simulink model "MSF_Proyecto_Angel_Montano_Rodriguez"  (R2024b)
settings: Solver=ode15s  StartTime=0.0  StopTime=10.0  MaxStep=1e-3  RelTol=1e-6  AbsTol=1e-10
libraries: fl_lib x18, nesl_utility x6, slpidlib x1
settings Model: Creator=ASUS  LastModifiedBy=ASUS
settings DataIOCC: SaveOutput=off  SignalLogging=off  DSMLogging=off  ReturnWorkspaceOutputs=off  TimeSaveName=t
settings DebuggingCC: AlgebraicLoopMsg=none  ArtificialAlgebraicLoopMsg=none  MaxConsecutiveZCsMsg=none  OperatingPointInterfaceChecksumMismatchMsg=none

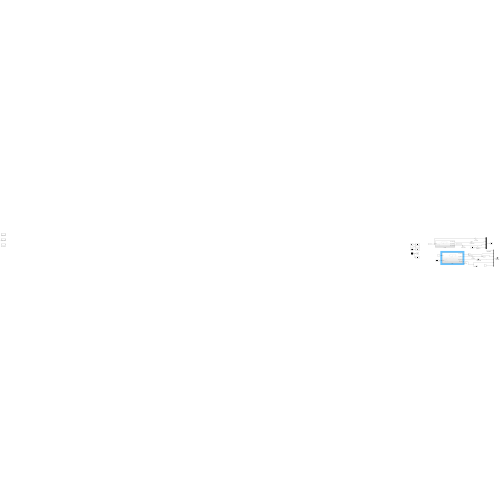
[thumbnail: Simulink's stored preview of the top-level diagram]
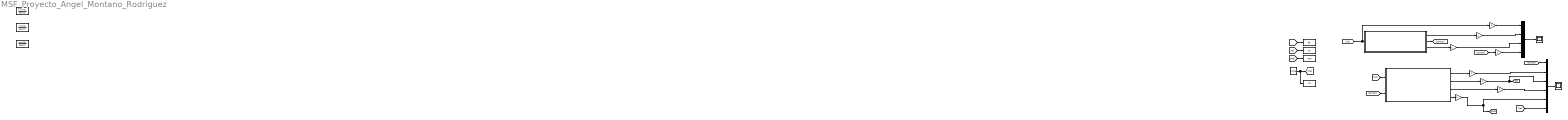
== system MSF_Proyecto_Angel_Montano_Rodriguez ==
  " Pp(t):Hipertenso" : TransferFcn  Numerator=[0.001,0.01]  Denominator=[0.00001,0.00101,0.01]
  " Pp(t):Hipotenso" : TransferFcn  Numerator=[0.001,0.01]  Denominator=[3.5E-5,0.00101,0.01]
  " Pp(t):Normotenso" : TransferFcn  Numerator=[0.001,0.01]  Denominator=[1.5E-5,0.00101,0.01]
  Caso : Subsystem
  Control : Subsystem
  EID(t): Control : Gain
  F(t): Caso CE : Gain
  F(t): Caso FT : Gain
  F(t): Control CE : Gain
  F(t): Control FT : Gain
  Mux2 : Mux  Inputs=6
  Mux3 : Mux
  PID(t): Caso : Gain
  Scope: Caso : Scope
  Scope: Control : Scope
  To Workspace1 : ToWorkspace  VariableName=Fe  SampleTime=-1
  To Workspace2 : ToWorkspace  VariableName=Fs  SampleTime=-1
  To Workspace3 : ToWorkspace  VariableName=PID  SampleTime=-1
  To Workspace4 : ToWorkspace  VariableName=Ve  SampleTime=-1
  Ve(t) : DiscretePulseGenerator  PulseType=Time based  Period=10  PulseWidth=10  PhaseDelay=1
  Ve(t) Control : Gain
  Ve(t): Caso EID : Gain
  wires:
  EID(t): Control/1 -> Mux3/3
  Mux3/1 -> Scope: Control/1
  F(t): Control CE/1 -> Mux3/2
  F(t): Control FT/1 -> Mux3/4
  F(t): Caso CE/1 -> Mux2/2
  Caso/1(Vs(t): Caso CE) -> F(t): Caso CE/1
  PID(t): Caso/1 -> Mux2/5, [PID]
  Mux2/1 -> Scope: Caso/1
  Caso/3(Ve(t): Caso EID) -> Ve(t): Caso EID/1
  Caso/4(PID(t): Caso) -> PID(t): Caso/1
  Ve(t)/1 -> To Workspace4/1, [Ve]
  [control] -> To Workspace1/1
  [Fs] -> To Workspace2/1
  [PID] -> To Workspace3/1
  Control/3(Ve(t): Control EID) -> EID(t): Control/1
  [control] -> F(t): Control FT/1
  Ve(t): Caso EID/1 -> Mux2/4
  Control/2(Ve(t): Control FT) -> [control]
  Control/1(Ve(t): Control CE) -> F(t): Control CE/1
  Caso/2(Ve(t): Caso FT) -> F(t): Caso FT/1
  [Ve] -> Ve(t) Control/1, Control/1(Ve(t))
  Ve(t) Control/1 -> Mux3/1
  [Ve] -> Caso/1(Vs(t))
  [control] -> Caso/2(Control)
  [Ve] -> Mux2/6
  [control] -> Mux2/1
  F(t): Caso FT/1 -> Mux2/3, [Fs]

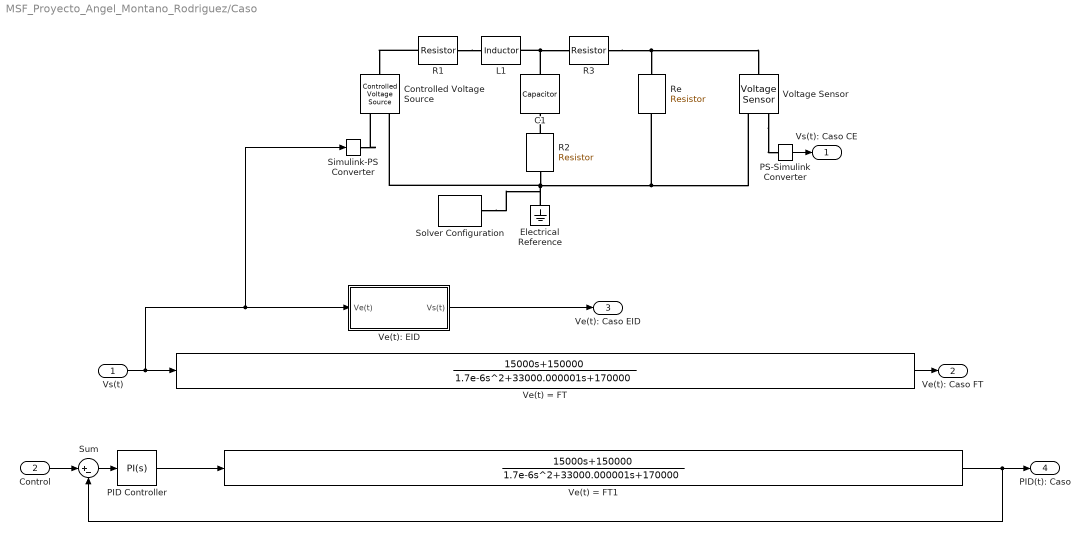
== system MSF_Proyecto_Angel_Montano_Rodriguez/Caso ==
  Vs(t) : Inport
  Control : Inport  Port=2
  " Ve(t) = FT" : TransferFcn  Numerator=[15000 150000]  Denominator=[1.7e-6 33000.000001 170000]
  " Ve(t) = FT1" : TransferFcn  Numerator=[15000 150000]  Denominator=[1.7e-6 33000.000001 170000]
  C1 : fl_lib/Electrical/Electrical Elements/Capacitor  c=10e-6 F  r=1e-6 Ohm  g=0 1/Ohm  i_specify=off  i_priority=None  i=0 A  i_nominal_specify=off  i_nominal_value=1  i_nominal_unit=A  v_specify=off  v_priority=None  v=0 V  v_nominal_specify=off  v_nominal_value=1  v_nominal_unit=V  vc_specify=off  vc_priority=High  vc=0 V  vc_nominal_specify=off  vc_nominal_value=1  vc_nominal_unit=V
  Controlled Voltage Source : fl_lib/Electrical/Electrical Sources/Controlled Voltage Source
  Electrical Reference : fl_lib/Electrical/Electrical Elements/Electrical Reference
  L1 : fl_lib/Electrical/Electrical Elements/Inductor  l=1e-6 H  r=0 Ohm  g=1e-9 1/Ohm  i_specify=off  i_priority=None  i=0 A  i_nominal_specify=off  i_nominal_value=1  i_nominal_unit=A  v_specify=off  v_priority=None  v=0 V  v_nominal_specify=off  v_nominal_value=1  v_nominal_unit=V  i_L_specify=off  i_L_priority=High  i_L=0 A  i_L_nominal_specify=off  i_L_nominal_value=1  i_L_nominal_unit=A
  PID Controller : slpidlib/PID Controller  Controller=PI  Form=Parallel  TimeDomain=Continuous-time  UseExternalTs=off  SampleTime=-1  IntegratorMethod=Forward Euler  FilterMethod=Forward Euler  ControllerParametersSource=internal  P=2  I=500  UseKiTs=off  D=0  UseExternalDerivativeSource=off  N=100  UseFilter=on  TunerSelectOption=Transfer Function Based (PID Tuner App)  InitialConditionSource=internal  InitialConditionForIntegrator=0  InitialConditionForFilter=0  DifferentiatorICPrevScaledInput=0  ExternalReset=none  TrackingMode=off  Kt=1  LimitOutput=off  SatLimitsSource=internal  UpperSaturationLimit=inf  LowerSaturationLimit=-inf  LinearizeAsGain=on  AntiWindupMode=none  Kb=1  LimitIntegrator=off  UpperIntegratorSaturationLimit=inf  LowerIntegratorSaturationLimit=-inf  POutMin=[]  POutMax=[]  IOutMin=[]  IOutMax=[]  DOutMin=[]  DOutMax=[]  NOutMin=[]  NOutMax=[]  SumOutMin=[]  SumOutMax=[]  SaturationOutMin=[]  SaturationOutMax=[]  PParamMin=[]  PParamMax=[]  IParamMin=[]  IParamMax=[]  DParamMin=[]  DParamMax=[]  NParamMin=[]  NParamMax=[]  KbParamMin=[]  KbParamMax=[]  KtParamMin=[]  KtParamMax=[]  KbOutMin=[]  KbOutMax=[]  KtOutMin=[]  KtOutMax=[]  IntegratorOutMin=[]  IntegratorOutMax=[]  FilterOutMin=[]  FilterOutMax=[]  SumI1OutMin=[]  SumI1OutMax=[]  SumI2OutMin=[]  SumI2OutMax=[]  SumI3OutMin=[]  SumI3OutMax=[]  SumI4OutMin=[]  SumI4OutMax=[]  SumDOutMin=[]  SumDOutMax=[]  DifferentiatorOutMin=[]  DifferentiatorOutMax=[]  FilterDiffOutCoefMin=[]  FilterDiffOutCoefMax=[]  ReciprocalOutMin=[]  ReciprocalOutMax=[]  SumDenOutMin=[]  SumDenOutMax=[]  SumNumOutMin=[]  SumNumOutMax=[]  DivideOutMin=[]  DivideOutMax=[]  UdiffTsProdOutMin=[]  UdiffTsProdOutMax=[]  NTsProdOutMin=[]  NTsProdOutMax=[]  UintegralTsProdOutMin=[]  UintegralTsProdOutMax=[]  UngainTsProdOutMin=[]  UngainTsProdOutMax=[]  ClampingZeroOutDataTypeStr=Inherit: Inherit via back propagation  ClampingZeroOutMin=[]  ClampingZeroOutMax=[]  FilterDenConstantOutDataTypeStr=Inherit: Inherit via back propagation  FilterDenConstantOutMin=[]  FilterDenConstantOutMax=[]  PCopyOutDataTypeStr=Inherit: Inherit via back propagation  PCopyOutMin=[]  PCopyOutMax=[]  NCopyOutDataTypeStr=Inherit: Inherit via back propagation  NCopyOutMin=[]  NCopyOutMax=[]  IntegratorContinuousStateAttributes=''  IntegratorStateMustResolveToSignalObject=off  IntegratorRTWStateStorageClass=Auto  FilterContinuousStateAttributes=''  FilterStateMustResolveToSignalObject=off  FilterRTWStateStorageClass=Auto  ParallelPVariant=InternalParameters  IdealPVariant=Disabled  IVariant=InternalParameters  DVariant=InternalParameters  IntegratorVariant=Continuous  SatVariant=Disabled  AWVariant=Passthrough  PCopyVariant=Disabled  TRVariant=Disabled  FdbkBlocksVariant=Forward  IdealPFdbkVariant=Disabled  SatFdbkVariant=Disabled  DerivativeFilterVariant=ContFilter  NVariant=InternalParameters  NCopyVariant=Disabled  FilterICVariant=InternalICsFilter  IntegratorICVariant=InternalICs  ExternalResetVariant=Disabled  TRSumVariant=Passthrough  SumFdbkVariant=Disabled  SumVariant=Sum_PID  TsampFilterVariant=InternalTs  TsampNgainVariant=Passthrough  TsampIntegralVariant=Disabled_SignalSpec  ExternalSaturationOutDataTypeStr=Inherit: Same as second input  DerivativeSourceVariant=ErrorSignal  PreIntVariant=InternalPreInt
  PS-Simulink Converter : nesl_utility/PS-Simulink Converter  PhysicalDomain=network_engine_domain  SubClassName=ps_output  LeftPortType=input  RightPortType=output  PseudoPeriodic=off  Frequencies=[]  VectorFormat=inherit  Unit=inherit  AffineConversion=off
  R1 : fl_lib/Electrical/Electrical Elements/Resistor  R=10 kOhm  i_specify=off  i_priority=None  i=0 A  i_nominal_specify=off  i_nominal_value=1  i_nominal_unit=A  v_specify=off  v_priority=None  v=0 V  v_nominal_specify=off  v_nominal_value=1  v_nominal_unit=V
  R2 : fl_lib/Electrical/Electrical Elements/Resistor  R=10 kOhm  i_specify=off  i_priority=None  i=0 A  i_nominal_specify=off  i_nominal_value=1  i_nominal_unit=A  v_specify=off  v_priority=None  v=0 V  v_nominal_specify=off  v_nominal_value=1  v_nominal_unit=V
  R3 : fl_lib/Electrical/Electrical Elements/Resistor  R=10 kOhm  i_specify=off  i_priority=None  i=0 A  i_nominal_specify=off  i_nominal_value=1  i_nominal_unit=A  v_specify=off  v_priority=None  v=0 V  v_nominal_specify=off  v_nominal_value=1  v_nominal_unit=V
  Re : fl_lib/Electrical/Electrical Elements/Resistor  R=150 kOhm  i_specify=off  i_priority=None  i=0 A  i_nominal_specify=off  i_nominal_value=1  i_nominal_unit=A  v_specify=off  v_priority=None  v=0 V  v_nominal_specify=off  v_nominal_value=1  v_nominal_unit=V
  Simulink-PS Converter : nesl_utility/Simulink-PS Converter  PhysicalDomain=network_engine_domain  SubClassName=ps_input  LeftPortType=input  RightPortType=output  PseudoPeriodic=off  Frequencies=[]  NoiseDistribution=none  NoiseParameters=[]  Unit=1  AffineConversion=off  FilteringAndDerivatives=provide  SimscapeFilterOrder=1  InputFilterTimeConstant=0.001  UdotUserProvided=0
  Solver Configuration : nesl_utility/Solver Configuration  PhysicalDomain=network_engine_domain  SubClassName=solver  LeftPortType=input  RightPortType=generic  Tones=[]  Harmonics=[]  SimulateNoise=off  Profile=off  UseLocalSampling=off  EnableSwitchedLinearOptims=on  FrequencyDomain=off  UseCCode=off  RelTol=0.001  AbsTol=0.001  MinStep=1e-09  ToWorkspace=off  RevertToSquareIcSolve=off  NumHomotopyIterations=100  PhasorMode=off  PhasorModeNumHarmonics=1  ConsistencySolver=NEWTON_XTOL_AFTER_FTOL  IndexReductionMethod=DerivativeReplacement  DoDC=off  ResidualTolerance=1e-09  ConsistencyTolSource=GLOBAL  ConsistencyAbsTol=0.001  ConsistencyRelTol=0.001  ConsistencyTolFactor=0.001  UseLocalSolver=off  LocalSolverChoice=NE_BACKWARD_EULER_ADVANCER  ResolveIndetEquations=on  FunctionEvalNumThread=1  LocalSolverSampleTime=0.001  DoFixedCost=off  MaxNonlinIter=3  MaxModeIter=2  ComputeImpulses=off  ImpulseIterations=2  LinearAlgebra=auto  LinearAlgebraNumThread=0  EquationFormulation=NE_TIME_EF  DelaysMemoryBudget=1024  AutomaticFiltering=on  FilteringTimeConstant=0.001  PartitionStorageMethod=AS_NEEDED  PartitionMemoryBudget=1024  PartitionMethod=ROBUST  MultibodyUseLocalSolver=off  MultibodyLocalSolverChoice=ODE1  MultibodyLocalSolverSampleTime=0.001
  Sum : Sum  Inputs=|+-
  Ve(t): EID : Subsystem
  Voltage Sensor : fl_lib/Electrical/Electrical Sensors/Voltage Sensor
  Vs(t): Caso CE : Outport
  Ve(t): Caso FT : Outport  Port=2
  Ve(t): Caso EID : Outport  Port=3
  PID(t): Caso : Outport  Port=4
  wires:
  PS-Simulink Converter/1 -> Vs(t): Caso CE/1
  Vs(t)/1 -> Ve(t): EID/1(Ve(t)), Simulink-PS Converter/1, " Ve(t) = FT"/1
  PID Controller/1 -> " Ve(t) = FT1"/1
  Control/1 -> Sum/1
  " Ve(t) = FT"/1 -> Ve(t): Caso FT/1
  Ve(t): EID/1(Vs(t)) -> Ve(t): Caso EID/1
  Sum/1 -> PID Controller/1
  " Ve(t) = FT1"/1 -> Sum/2, PID(t): Caso/1
  connections:
  C1/LConn1 -- R3/LConn1 -- L1/RConn1
  R2/RConn1 -- Solver Configuration/RConn1 -- Electrical Reference/LConn1 -- Controlled Voltage Source/RConn2 -- Voltage Sensor/RConn2 -- Re/RConn1
  R3/RConn1 -- Voltage Sensor/LConn1 -- Re/LConn1
  Voltage Sensor/RConn1 -- PS-Simulink Converter/LConn1
  R1/RConn1 -- L1/LConn1
  Simulink-PS Converter/RConn1 -- Controlled Voltage Source/RConn1
  R2/LConn1 -- C1/RConn1
  R1/LConn1 -- Controlled Voltage Source/LConn1

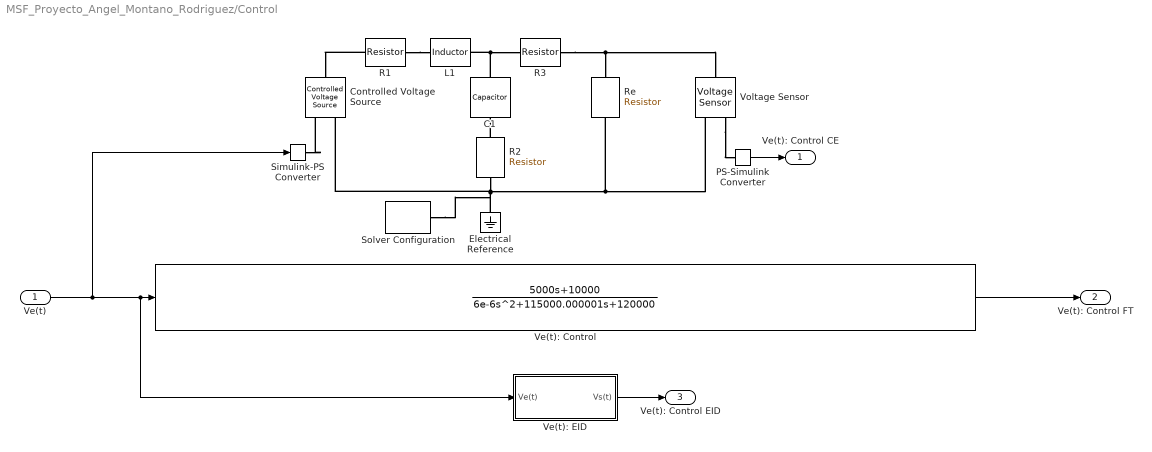
== system MSF_Proyecto_Angel_Montano_Rodriguez/Control ==
  Ve(t) : Inport
  " Ve(t): Control" : TransferFcn  Numerator=[5000 10000]  Denominator=[6e-6 115000.000001 120000]
  C1 : fl_lib/Electrical/Electrical Elements/Capacitor  c=50e-6 F  r=1e-6 Ohm  g=0 1/Ohm  i_specify=off  i_priority=None  i=0 A  i_nominal_specify=off  i_nominal_value=1  i_nominal_unit=A  v_specify=off  v_priority=None  v=0 V  v_nominal_specify=off  v_nominal_value=1  v_nominal_unit=V  vc_specify=off  vc_priority=High  vc=0 V  vc_nominal_specify=off  vc_nominal_value=1  vc_nominal_unit=V
  Controlled Voltage Source : fl_lib/Electrical/Electrical Sources/Controlled Voltage Source
  Electrical Reference : fl_lib/Electrical/Electrical Elements/Electrical Reference
  L1 : fl_lib/Electrical/Electrical Elements/Inductor  l=1e-6 H  r=0 Ohm  g=1e-9 1/Ohm  i_specify=off  i_priority=None  i=0 A  i_nominal_specify=off  i_nominal_value=1  i_nominal_unit=A  v_specify=off  v_priority=None  v=0 V  v_nominal_specify=off  v_nominal_value=1  v_nominal_unit=V  i_L_specify=off  i_L_priority=High  i_L=0 A  i_L_nominal_specify=off  i_L_nominal_value=1  i_L_nominal_unit=A
  PS-Simulink Converter : nesl_utility/PS-Simulink Converter  PhysicalDomain=network_engine_domain  SubClassName=ps_output  LeftPortType=input  RightPortType=output  PseudoPeriodic=off  Frequencies=[]  VectorFormat=inherit  Unit=inherit  AffineConversion=off
  R1 : fl_lib/Electrical/Electrical Elements/Resistor  R=10 kOhm  i_specify=off  i_priority=None  i=0 A  i_nominal_specify=off  i_nominal_value=1  i_nominal_unit=A  v_specify=off  v_priority=None  v=0 V  v_nominal_specify=off  v_nominal_value=1  v_nominal_unit=V
  R2 : fl_lib/Electrical/Electrical Elements/Resistor  R=10 kOhm  i_specify=off  i_priority=None  i=0 A  i_nominal_specify=off  i_nominal_value=1  i_nominal_unit=A  v_specify=off  v_priority=None  v=0 V  v_nominal_specify=off  v_nominal_value=1  v_nominal_unit=V
  R3 : fl_lib/Electrical/Electrical Elements/Resistor  R=100 kOhm  i_specify=off  i_priority=None  i=0 A  i_nominal_specify=off  i_nominal_value=1  i_nominal_unit=A  v_specify=off  v_priority=None  v=0 V  v_nominal_specify=off  v_nominal_value=1  v_nominal_unit=V
  Re : fl_lib/Electrical/Electrical Elements/Resistor  R=10 kOhm  i_specify=off  i_priority=None  i=0 A  i_nominal_specify=off  i_nominal_value=1  i_nominal_unit=A  v_specify=off  v_priority=None  v=0 V  v_nominal_specify=off  v_nominal_value=1  v_nominal_unit=V
  Simulink-PS Converter : nesl_utility/Simulink-PS Converter  PhysicalDomain=network_engine_domain  SubClassName=ps_input  LeftPortType=input  RightPortType=output  PseudoPeriodic=off  Frequencies=[]  NoiseDistribution=none  NoiseParameters=[]  Unit=1  AffineConversion=off  FilteringAndDerivatives=provide  SimscapeFilterOrder=1  InputFilterTimeConstant=0.001  UdotUserProvided=0
  Solver Configuration : nesl_utility/Solver Configuration  PhysicalDomain=network_engine_domain  SubClassName=solver  LeftPortType=input  RightPortType=generic  Tones=[]  Harmonics=[]  SimulateNoise=off  Profile=off  UseLocalSampling=off  EnableSwitchedLinearOptims=on  FrequencyDomain=off  UseCCode=off  RelTol=0.001  AbsTol=0.001  MinStep=1e-09  ToWorkspace=off  RevertToSquareIcSolve=off  NumHomotopyIterations=100  PhasorMode=off  PhasorModeNumHarmonics=1  ConsistencySolver=NEWTON_XTOL_AFTER_FTOL  IndexReductionMethod=DerivativeReplacement  DoDC=off  ResidualTolerance=1e-09  ConsistencyTolSource=GLOBAL  ConsistencyAbsTol=0.001  ConsistencyRelTol=0.001  ConsistencyTolFactor=0.001  UseLocalSolver=off  LocalSolverChoice=NE_BACKWARD_EULER_ADVANCER  ResolveIndetEquations=on  FunctionEvalNumThread=1  LocalSolverSampleTime=0.001  DoFixedCost=off  MaxNonlinIter=3  MaxModeIter=2  ComputeImpulses=off  ImpulseIterations=2  LinearAlgebra=auto  LinearAlgebraNumThread=0  EquationFormulation=NE_TIME_EF  DelaysMemoryBudget=1024  AutomaticFiltering=on  FilteringTimeConstant=0.001  PartitionStorageMethod=AS_NEEDED  PartitionMemoryBudget=1024  PartitionMethod=ROBUST  MultibodyUseLocalSolver=off  MultibodyLocalSolverChoice=ODE1  MultibodyLocalSolverSampleTime=0.001
  Ve(t): EID : Subsystem
  Voltage Sensor : fl_lib/Electrical/Electrical Sensors/Voltage Sensor
  Ve(t): Control CE : Outport
  Ve(t): Control FT : Outport  Port=2
  Ve(t): Control EID : Outport  Port=3
  wires:
  PS-Simulink Converter/1 -> Ve(t): Control CE/1
  Ve(t)/1 -> Ve(t): EID/1(Ve(t)), " Ve(t): Control"/1, Simulink-PS Converter/1
  " Ve(t): Control"/1 -> Ve(t): Control FT/1
  Ve(t): EID/1(Vs(t)) -> Ve(t): Control EID/1
  connections:
  R2/RConn1 -- Solver Configuration/RConn1 -- Electrical Reference/LConn1 -- Controlled Voltage Source/RConn2 -- Voltage Sensor/RConn2 -- Re/RConn1
  R3/RConn1 -- Voltage Sensor/LConn1 -- Re/LConn1
  C1/LConn1 -- R3/LConn1 -- L1/RConn1
  Voltage Sensor/RConn1 -- PS-Simulink Converter/LConn1
  R1/LConn1 -- Controlled Voltage Source/LConn1
  Simulink-PS Converter/RConn1 -- Controlled Voltage Source/RConn1
  R1/RConn1 -- L1/LConn1
  R2/LConn1 -- C1/RConn1

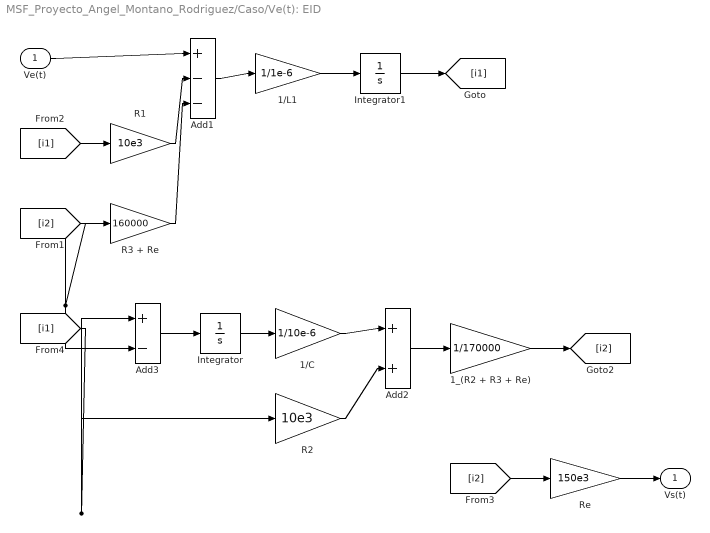
== system MSF_Proyecto_Angel_Montano_Rodriguez/Caso/Ve(t): EID ==
  Ve(t) : Inport
  1/C : Gain  Gain=1/10e-6
  1/L1 : Gain  Gain=1/1e-6
  1_(R2 + R3 + Re) : Gain  Gain=1/170000
  Add1 : Sum  Inputs=+--
  Add2 : Sum
  Add3 : Sum  Inputs=+-
  Integrator : Integrator
  Integrator1 : Integrator
  R1 : Gain  Gain=10e3
  R2 : Gain  Gain=10e3
  R3 + Re : Gain  Gain=160000
  Re : Gain  Gain=150e3
  Vs(t) : Outport
  wires:
  Ve(t)/1 -> Add1/1
  [i1] -> R1/1
  R1/1 -> Add1/2
  [i2] -> R3 + Re/1, Add3/2
  R3 + Re/1 -> Add1/3
  Add1/1 -> 1/L1/1
  1/L1/1 -> Integrator1/1
  Integrator1/1 -> [i1]
  [i1] -> Add3/1, R2/1
  Add3/1 -> Integrator/1
  Integrator/1 -> 1/C/1
  1/C/1 -> Add2/1
  R2/1 -> Add2/2
  Add2/1 -> 1_(R2 + R3 + Re)/1
  1_(R2 + R3 + Re)/1 -> [i2]
  [i2] -> Re/1
  Re/1 -> Vs(t)/1

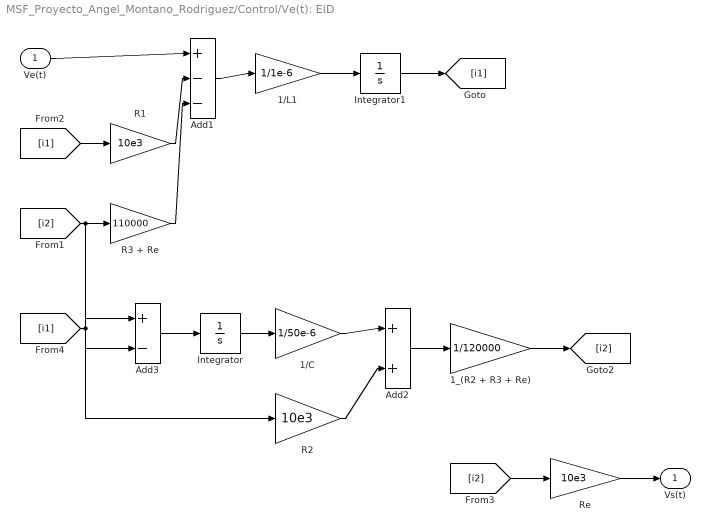
== system MSF_Proyecto_Angel_Montano_Rodriguez/Control/Ve(t): EID ==
  Ve(t) : Inport
  1/C : Gain  Gain=1/50e-6
  1/L1 : Gain  Gain=1/1e-6
  1_(R2 + R3 + Re) : Gain  Gain=1/120000
  Add1 : Sum  Inputs=+--
  Add2 : Sum
  Add3 : Sum  Inputs=+-
  Integrator : Integrator
  Integrator1 : Integrator
  R1 : Gain  Gain=10e3
  R2 : Gain  Gain=10e3
  R3 + Re : Gain  Gain=110000
  Re : Gain  Gain=10e3
  Vs(t) : Outport
  wires:
  Ve(t)/1 -> Add1/1
  [i1] -> R1/1
  R1/1 -> Add1/2
  [i2] -> R3 + Re/1, Add3/2
  R3 + Re/1 -> Add1/3
  Add1/1 -> 1/L1/1
  1/L1/1 -> Integrator1/1
  Integrator1/1 -> [i1]
  [i1] -> Add3/1, R2/1
  Add3/1 -> Integrator/1
  Integrator/1 -> 1/C/1
  1/C/1 -> Add2/1
  R2/1 -> Add2/2
  Add2/1 -> 1_(R2 + R3 + Re)/1
  1_(R2 + R3 + Re)/1 -> [i2]
  [i2] -> Re/1
  Re/1 -> Vs(t)/1
